simulink model "HybridFusionTest"  (R2026b)
settings: Solver=FixedStepDiscrete  StopTime=fusionTestCfg.Duration  FixedStep=fusionCfg.Ts
PostLoadFcn:
  | addpath(fullfile(fileparts(get_param(bdroot,'FileName')),'..','build_process'));initialize_hybrid_fusion_test(bdroot);
model workspace (MAT data in the model file):
  fusionCfg.Ts = 5e-05
  fusionCfg.LowOmega = 40
  fusionCfg.HighOmega = 60
  fusionCfg.LowMaxOmega = 80
  fusionCfg.HighMinOmega = 30
  fusionCfg.MaxPhaseGap = 0.7
  fusionCfg.MaxSpeedGap = 30
  fusionCfg.QualificationTime = 0.01
  fusionCfg.LossTime = 0.002
  fusionCfg.BlendTime = 0.05
  fusionCfg.InjectionRampTime = 0.02
  fusionCfg.InjectionResumeOmega = 65
  fusionCfg.InjectionOffOmega = 75
  fusionCfg.PhaseCorrectionRate = 20
  fusionCfg.MaxPhaseInnovation = 0.2
  fusionCfg.MinInjectionScale = 0.1
  fusionCfg.AllowHighStart = 1
  fusionCfg.QualificationSamples = 200
  fusionCfg.LossSamples = 40
  fusionCfg.Vector = [5e-05; 40; 60; 80; 0.7; 30; 200; 40; 0.001; 0.0025; 65; 75; 20; 0.2; 1; 30; 0.1]
  fusionCfg.State0 = [0; 0; 0; 1; 0; 0; 0; 0; 0; 0; 0; 0; 0; 0; 0; 0; 0; 1; 0; 0]
  fusionTestCfg.Duration = 1.3
  fusionTestCfg.InitialAngle = 0.3
  fusionTestCfg.InitialOmega = 20
  fusionTestCfg.PeakOmega = 100
  fusionTestCfg.RampStart = 0.1
  fusionTestCfg.RampEnd = 0.5
  fusionTestCfg.DownStart = 0.7
  fusionTestCfg.DownEnd = 1.1
  fusionTestCfg.LowPhaseBias = -0.03
  fusionTestCfg.HighPhaseBias = 0.02
  fusionTestCfg.ReturnPi = 1
  fusionTestCfg.ReturnTime = 0.85
  fusionTestCfg.Enable = 1
  fusionTestCfg.Reset = 0
  testStim.time = [0 5e-05 0.0001 0.00015 0.0002 0.00025 0.0003 0.00035 0.0004 0.00045 0.0005 0.00055 ... (26001 elements, 26001x1)]
  testStim.signals.values = [0.27 0.271 0.272 0.273 0.274 0.275 0.276 0.277 0.278 0.279 0.28 0.281 ... (260010 elements, 26001x10)]
  testStim.signals.dimensions = 10
libraries: SensorlessHandover x1
settings Model: Creator=24322  LastModifiedBy=24322

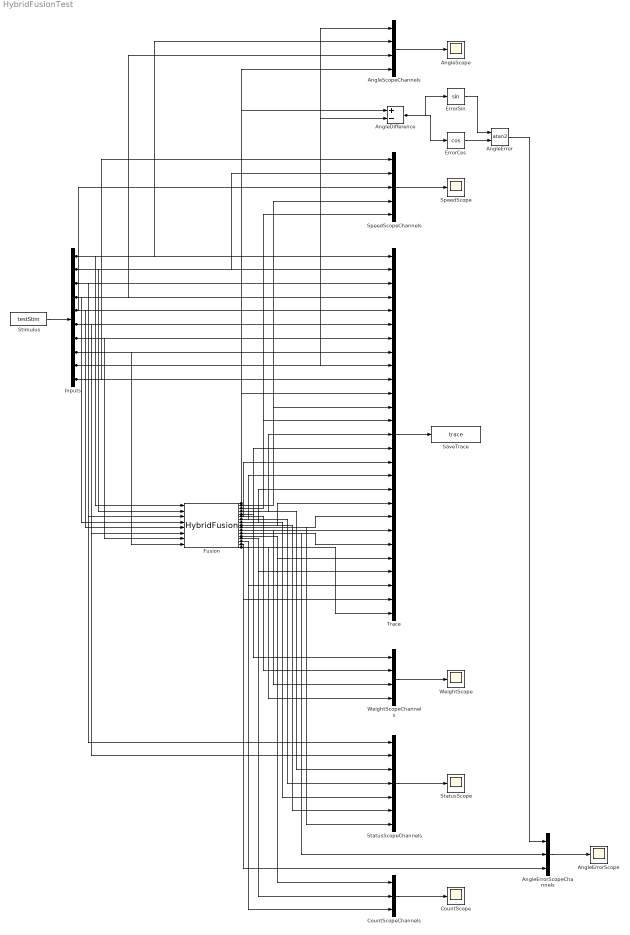
== system HybridFusionTest ==
  AngleDifference : Sum  Inputs=+-
  AngleError : Trigonometry  Operator=atan2
  AngleErrorScope : Scope
  AngleErrorScopeChannels : Mux  Inputs=3
  AngleScope : Scope
  AngleScopeChannels : Mux
  CountScope : Scope
  CountScopeChannels : Mux  Inputs=3
  ErrorCos : Trigonometry  Operator=cos
  ErrorSin : Trigonometry
  Fusion : SensorlessHandover/HybridFusion  fusionCfg=fusionCfg
  Inputs : Demux  Outputs=10
  SaveTrace : ToWorkspace  VariableName=trace  SaveFormat=Structure With Time  SampleTime=fusionCfg.Ts
  SpeedScope : Scope
  SpeedScopeChannels : Mux  Inputs=5
  StatusScope : Scope
  StatusScopeChannels : Mux  Inputs=7
  Stimulus : FromWorkspace  VariableName=testStim  SampleTime=fusionCfg.Ts  Interpolate=off  OutputAfterFinalValue=Holding final value
  Trace : Mux  Inputs=27
  WeightScope : Scope
  WeightScopeChannels : Mux
  wires:
  CountScopeChannels/1 -> CountScope/1
  StatusScopeChannels/1 -> StatusScope/1
  WeightScopeChannels/1 -> WeightScope/1
  SpeedScopeChannels/1 -> SpeedScope/1
  AngleError/1 -> AngleErrorScopeChannels/1
  AngleErrorScopeChannels/1 -> AngleErrorScope/1
  AngleScopeChannels/1 -> AngleScope/1
  Fusion/17 -> Trace/27, WeightScopeChannels/4
  Fusion/16 -> Trace/26, AngleErrorScopeChannels/3
  Fusion/15 -> Trace/25, CountScopeChannels/3
  Fusion/14 -> Trace/24, CountScopeChannels/2
  Fusion/13 -> Trace/23, CountScopeChannels/1
  Fusion/12 -> Trace/22, AngleErrorScopeChannels/2
  Fusion/11 -> Trace/21, WeightScopeChannels/3
  Fusion/10 -> Trace/20, StatusScopeChannels/7
  Fusion/9 -> Trace/19, StatusScopeChannels/6
  Fusion/8 -> Trace/18, StatusScopeChannels/5
  Fusion/7 -> Trace/17, StatusScopeChannels/4
  Fusion/6 -> Trace/16, WeightScopeChannels/2
  Fusion/5 -> Trace/15, WeightScopeChannels/1
  Fusion/4 -> Trace/14, StatusScopeChannels/3
  Fusion/3 -> Trace/13, SpeedScopeChannels/5
  Fusion/2 -> Trace/12, SpeedScopeChannels/4
  Inputs/10 -> Trace/10, SpeedScopeChannels/1
  Inputs/8 -> Trace/8, Fusion/8
  Inputs/7 -> Trace/7, Fusion/7
  Inputs/6 -> Fusion/6, Trace/6, StatusScopeChannels/2
  Inputs/5 -> Trace/5, Fusion/5, SpeedScopeChannels/3
  Inputs/4 -> Fusion/4, Trace/4, AngleScopeChannels/3
  Inputs/3 -> Fusion/3, Trace/3, StatusScopeChannels/1
  Inputs/2 -> Fusion/2, Trace/2, SpeedScopeChannels/2
  Inputs/1 -> Fusion/1, Trace/1, AngleScopeChannels/2
  ErrorCos/1 -> AngleError/2
  ErrorSin/1 -> AngleError/1
  AngleDifference/1 -> ErrorSin/1, ErrorCos/1
  Inputs/9 -> Trace/9, AngleDifference/2, AngleScopeChannels/1
  Fusion/1 -> AngleDifference/1, Trace/11, AngleScopeChannels/4
  Trace/1 -> SaveTrace/1
  Stimulus/1 -> Inputs/1
